simulink model "WBR_Simulator"  (R2023b)
settings: Solver=FixedStepAuto  StartTime=0.0  StopTime=60  FixedStep=0.001  MaxStep=0.001
undefined symbols (not defined in the file or in its folder): DiscIntNeverNeededParam, magnitude, robot_stats, SIMPARAM, X, Y, Z
libraries: sm_lib x73, nesl_utility x50, simulink x17, slpidlib x6, dsparch4 x2
(part 3 of 7)

== system WBR_Simulator/轮子建模 ==
  note: 左轮
  note: 右轮
  左轮控制扭矩 : Inport
  右轮控制扭矩 : Inport  Port=2
  Brick Solid : sm_lib/Body Elements/Brick Solid  GraphicAmbientColor=[0.15 0.15 0.15 1.0]  BasedOnType=Mass  BrickDimensions=[0.1 0.05 0.1]  BrickDimensionsUnits=m  CenterOfMass=[0 0 0]  CenterOfMassUnits=m  GraphicDiffuseColor=[0.5 0.5 0.5]  Density=1000  DensityUnits=kg/m^3  DoExposeReferenceFrame=on  GraphicEmissiveColor=[0.0 0.0 0.0 1.0]  ExportEntireGeometry=off  SerializedFrames=<Frames/>  MarkerShape=Sphere  MarkerSize=10  GraphicType=FromGeometry  InertiaType=CalculateFromGeometry  Mass=0.000001  MassUnits=kg  MomentsOfInertia=[1 1 1]  MomentsOfInertiaUnits=kg*m^2  GraphicOpacity=1.0  ProductsOfInertia=[0 0 0]  ProductsOfInertiaUnits=kg*m^2  GraphicShininess=75  GraphicSpecularColor=[0.5 0.5 0.5 1.0]  GraphicVisPropType=SimpleVisualProperties
  Brick Solid1 : sm_lib/Body Elements/Brick Solid  GraphicAmbientColor=[0.15 0.15 0.15 1.0]  BasedOnType=Mass  BrickDimensions=[0.1 0.05 0.1]  BrickDimensionsUnits=m  CenterOfMass=[0 0 0]  CenterOfMassUnits=m  GraphicDiffuseColor=[0.5 0.5 0.5]  Density=1000  DensityUnits=kg/m^3  DoExposeReferenceFrame=on  GraphicEmissiveColor=[0.0 0.0 0.0 1.0]  ExportEntireGeometry=off  SerializedFrames=<Frames/>  MarkerShape=Sphere  MarkerSize=10  GraphicType=FromGeometry  InertiaType=CalculateFromGeometry  Mass=0.000001  MassUnits=kg  MomentsOfInertia=[1 1 1]  MomentsOfInertiaUnits=kg*m^2  GraphicOpacity=1.0  ProductsOfInertia=[0 0 0]  ProductsOfInertiaUnits=kg*m^2  GraphicShininess=75  GraphicSpecularColor=[0.5 0.5 0.5 1.0]  GraphicVisPropType=SimpleVisualProperties
  Bus Creator3 : BusCreator  Inputs=4
  Cylindrical Solid : sm_lib/Body Elements/Cylindrical Solid  GraphicAmbientColor=[0.15 0.15 0.15 1.0]  BasedOnType=Mass  CenterOfMass=[0 0 0]  CenterOfMassUnits=m  GraphicDiffuseColor=[0.0 0.4 0.4]  CylinderLength=0.05  CylinderLengthUnits=m  CylinderRadius=robot_stats.radius_wheel  CylinderRadiusUnits=m  Density=1000  DensityUnits=kg/m^3  DoExposeReferenceFrame=off  GraphicEmissiveColor=[0.0 0.0 0.0 1.0]  ExportEntireGeometry=on  SerializedFrames=<Frames><Frame><Id>Frame1</Id><Value><Name>center</Name><Origin><Source>GeometricFeature</Source><FeatureName>bottom surface</FeatureName></Origin><PrimaryAxis><DefinedDirection>+Z</DefinedDirection><Source>ReferenceFrame</Source><SourceDirection>+Z</SourceDirection><FeatureName></FeatureName></PrimaryAxis><SecondaryAxis><DefinedDirection>+X</DefinedDirection><Source>ReferenceFrame</Source><SourceDirection>+X</SourceDirection><FeatureName></FeatureName></SecondaryAxis></Value></Frame><Frame><Id>Frame2</Id><Value><Name>F2</Name><Origin><Source>CenterOfMassFrame</Source><FeatureName></FeatureName></Origin><PrimaryAxis><DefinedDirection>+Z</DefinedDirection><Source>ReferenceFrame</Source><SourceDirection>+Z</SourceDirection><FeatureName></FeatureName></PrimaryAxis><SecondaryAxis><DefinedDirection>+X</DefinedDirection><Source>ReferenceFrame</Source><SourceDirection>+X</SourceDirection><FeatureName></FeatureName></SecondaryAxis></Value></Frame></Frames>  MarkerShape=Sphere  MarkerSize=10  GraphicType=FromGeometry  InertiaType=CalculateFromGeometry  Mass=robot_stats.mass_wheel_aver/2  MassUnits=kg  MomentsOfInertia=[1 1 1]  MomentsOfInertiaUnits=kg*m^2  GraphicOpacity=1.0  ProductsOfInertia=[0 0 0]  ProductsOfInertiaUnits=kg*m^2  GraphicShininess=75  GraphicSpecularColor=[0.5 0.5 0.5 1.0]  GraphicVisPropType=SimpleVisualProperties
  Cylindrical Solid1 : sm_lib/Body Elements/Cylindrical Solid  GraphicAmbientColor=[0.15 0.15 0.15 1.0]  BasedOnType=Mass  CenterOfMass=[0 0 0]  CenterOfMassUnits=m  GraphicDiffuseColor=[0.0 0.4 0.4]  CylinderLength=0.05  CylinderLengthUnits=m  CylinderRadius=robot_stats.radius_wheel  CylinderRadiusUnits=m  Density=1000  DensityUnits=kg/m^3  DoExposeReferenceFrame=off  GraphicEmissiveColor=[0.0 0.0 0.0 1.0]  ExportEntireGeometry=on  SerializedFrames=<Frames><Frame><Id>Frame1</Id><Value><Name>center</Name><Origin><Source>GeometricFeature</Source><FeatureName>top surface</FeatureName></Origin><PrimaryAxis><DefinedDirection>+Z</DefinedDirection><Source>ReferenceFrame</Source><SourceDirection>+Z</SourceDirection><FeatureName></FeatureName></PrimaryAxis><SecondaryAxis><DefinedDirection>+X</DefinedDirection><Source>ReferenceFrame</Source><SourceDirection>+X</SourceDirection><FeatureName></FeatureName></SecondaryAxis></Value></Frame><Frame><Id>Frame2</Id><Value><Name>F2</Name><Origin><Source>CenterOfMassFrame</Source><FeatureName></FeatureName></Origin><PrimaryAxis><DefinedDirection>+Z</DefinedDirection><Source>ReferenceFrame</Source><SourceDirection>+Z</SourceDirection><FeatureName></FeatureName></PrimaryAxis><SecondaryAxis><DefinedDirection>+X</DefinedDirection><Source>ReferenceFrame</Source><SourceDirection>+X</SourceDirection><FeatureName></FeatureName></SecondaryAxis></Value></Frame></Frames>  MarkerShape=Sphere  MarkerSize=10  GraphicType=FromGeometry  InertiaType=CalculateFromGeometry  Mass=robot_stats.mass_wheel_aver/2  MassUnits=kg  MomentsOfInertia=[1 1 1]  MomentsOfInertiaUnits=kg*m^2  GraphicOpacity=1.0  ProductsOfInertia=[0 0 0]  ProductsOfInertiaUnits=kg*m^2  GraphicShininess=75  GraphicSpecularColor=[0.5 0.5 0.5 1.0]  GraphicVisPropType=SimpleVisualProperties
  Discrete-Time Integrator : DiscreteIntegrator  SampleTime=-1  ICPrevOutput=DiscIntNeverNeededParam  ICPrevScaledInput=DiscIntNeverNeededParam
  Discrete-Time Integrator1 : DiscreteIntegrator  SampleTime=-1  ICPrevOutput=DiscIntNeverNeededParam  ICPrevScaledInput=DiscIntNeverNeededParam
  Multiply : Gain  Gain=robot_stats.radius_wheel
  Multiply1 : Gain  Gain=robot_stats.radius_wheel
  PS-Simulink Converter : nesl_utility/PS-Simulink Converter  PhysicalDomain=network_engine_domain  SubClassName=ps_output  LeftPortType=input  RightPortType=output  PseudoPeriodic=off  Frequencies=[]  VectorFormat=1-D array  Unit=inherit  AffineConversion=off
  PS-Simulink Converter2 : nesl_utility/PS-Simulink Converter  PhysicalDomain=network_engine_domain  SubClassName=ps_output  LeftPortType=input  RightPortType=output  PseudoPeriodic=off  Frequencies=[]  VectorFormat=1-D array  Unit=inherit  AffineConversion=off
  Revolute Joint2 : sm_lib/Joints/Revolute Joint  JointMode=Normal  SenseConstraintForce=off  SenseConstraintForceX=off  SenseConstraintForceY=off  SenseConstraintForceZ=off  SenseConstraintTorque=off  SenseConstraintTorqueX=off  SenseConstraintTorqueY=off  SenseConstraintTorqueZ=off  SenseTotalForce=off  SenseTotalForceX=off  SenseTotalForceY=off  SenseTotalForceZ=off  SenseTotalTorque=off  SenseTotalTorqueX=off  SenseTotalTorqueY=off  SenseTotalTorqueZ=off  CompositeWrenchDir=FollowerOnBase  CompositeWrenchFrame=BaseFrame  EquilibriumPosition=0  EquilibriumPositionUnits=deg  SpringStiffness=0  SpringStiffnessUnits=N*m/deg  DampingCoefficient=0  DampingCoefficientUnits=N*m/(deg/s)  TorqueActuationMode=InputTorque  MotionActuationMode=ComputedMotion  SensePosition=off  SenseVelocity=on  SenseAcceleration=off  SenseTorqueForce=off  SenseLowerLimitTorqueForce=off  SenseUpperLimitTorqueForce=off  LowerLimitSpecify=off  LowerLimitBound=-90  LowerLimitBoundUnits=deg  LowerLimitStiffness=1e4  LowerLimitStiffnessUnits=N*m/deg  LowerLimitDamping=10  LowerLimitDampingUnits=N*m/(deg/s)  LowerLimitTransitionRegionWidth=0.1  LowerLimitTransitionRegionWidthUnits=deg  UpperLimitSpecify=off  UpperLimitBound=90  UpperLimitBoundUnits=deg  UpperLimitStiffness=1e4  UpperLimitStiffnessUnits=N*m/deg  UpperLimitDamping=10  UpperLimitDampingUnits=N*m/(deg/s)  UpperLimitTransitionRegionWidth=0.1  UpperLimitTransitionRegionWidthUnits=deg  PositionTargetSpecify=on  PositionTargetPriority=High  PositionTargetValue=0  PositionTargetValueUnits=deg  VelocityTargetSpecify=off  VelocityTargetPriority=High  VelocityTargetValue=0  VelocityTargetValueUnits=deg/s
  Revolute Joint7 : sm_lib/Joints/Revolute Joint  JointMode=Normal  SenseConstraintForce=off  SenseConstraintForceX=off  SenseConstraintForceY=off  SenseConstraintForceZ=off  SenseConstraintTorque=off  SenseConstraintTorqueX=off  SenseConstraintTorqueY=off  SenseConstraintTorqueZ=off  SenseTotalForce=off  SenseTotalForceX=off  SenseTotalForceY=off  SenseTotalForceZ=off  SenseTotalTorque=off  SenseTotalTorqueX=off  SenseTotalTorqueY=off  SenseTotalTorqueZ=off  CompositeWrenchDir=FollowerOnBase  CompositeWrenchFrame=BaseFrame  EquilibriumPosition=0  EquilibriumPositionUnits=deg  SpringStiffness=0  SpringStiffnessUnits=N*m/deg  DampingCoefficient=0  DampingCoefficientUnits=N*m/(deg/s)  TorqueActuationMode=InputTorque  MotionActuationMode=ComputedMotion  SensePosition=off  SenseVelocity=on  SenseAcceleration=off  SenseTorqueForce=off  SenseLowerLimitTorqueForce=off  SenseUpperLimitTorqueForce=off  LowerLimitSpecify=off  LowerLimitBound=-90  LowerLimitBoundUnits=deg  LowerLimitStiffness=1e4  LowerLimitStiffnessUnits=N*m/deg  LowerLimitDamping=10  LowerLimitDampingUnits=N*m/(deg/s)  LowerLimitTransitionRegionWidth=0.1  LowerLimitTransitionRegionWidthUnits=deg  UpperLimitSpecify=off  UpperLimitBound=90  UpperLimitBoundUnits=deg  UpperLimitStiffness=1e4  UpperLimitStiffnessUnits=N*m/deg  UpperLimitDamping=10  UpperLimitDampingUnits=N*m/(deg/s)  UpperLimitTransitionRegionWidth=0.1  UpperLimitTransitionRegionWidthUnits=deg  PositionTargetSpecify=on  PositionTargetPriority=High  PositionTargetValue=0  PositionTargetValueUnits=deg  VelocityTargetSpecify=off  VelocityTargetPriority=High  VelocityTargetValue=0  VelocityTargetValueUnits=deg/s
  Rigid Transform : sm_lib/Frames and Transforms/Rigid Transform  TranslationMethod=Cartesian  TranslationStandardOffset=1.5  TranslationStandardOffsetUnits=m  TranslationStandardAxis=-X  TranslationCartesianOffset=[0 0 0]  TranslationCartesianOffsetUnits=m  TranslationROffset=0  TranslationROffsetUnits=m  TranslationZOffset=0  TranslationZOffsetUnits=m  TranslationThetaOffset=0  TranslationThetaOffsetUnits=deg  RotationMethod=StandardAxis  RotationAngleUnits=deg  RotationStandardAxis=+Y  RotationAngle=0  RotationArbitraryAxis=[0 0 1]  FollAlignAxisA=+X  BaseAlignAxisA=+Y  FollAlignAxisB=+Y  BaseAlignAxisB=+Z  RotationSequenceAxes=FollowerAxes  RotationSequence=XYX  RotationSequenceAngles=[0 0 0]  RotationSequenceAnglesUnits=deg  RotationMatrix=[1 0 0; 0 1 0; 0 0 1]  Quaternion=[1 0 0 0]
  Rigid Transform1 : sm_lib/Frames and Transforms/Rigid Transform  TranslationMethod=Cartesian  TranslationStandardOffset=1.5  TranslationStandardOffsetUnits=m  TranslationStandardAxis=-X  TranslationCartesianOffset=[0 0 0]  TranslationCartesianOffsetUnits=m  TranslationROffset=0  TranslationROffsetUnits=m  TranslationZOffset=0  TranslationZOffsetUnits=m  TranslationThetaOffset=0  TranslationThetaOffsetUnits=deg  RotationMethod=StandardAxis  RotationAngleUnits=deg  RotationStandardAxis=+Y  RotationAngle=0  RotationArbitraryAxis=[0 0 1]  FollAlignAxisA=+X  BaseAlignAxisA=+Y  FollAlignAxisB=+Y  BaseAlignAxisB=+Z  RotationSequenceAxes=FollowerAxes  RotationSequence=XYX  RotationSequenceAngles=[0 0 0]  RotationSequenceAnglesUnits=deg  RotationMatrix=[1 0 0; 0 1 0; 0 0 1]  Quaternion=[1 0 0 0]
  Simulink-PS Converter : nesl_utility/Simulink-PS Converter  PhysicalDomain=network_engine_domain  SubClassName=ps_input  LeftPortType=input  RightPortType=output  PseudoPeriodic=off  Frequencies=[]  NoiseDistribution=none  NoiseParameters=[]  Unit=1  AffineConversion=off  FilteringAndDerivatives=provide  SimscapeFilterOrder=1  InputFilterTimeConstant=0.001  UdotUserProvided=0
  Simulink-PS Converter1 : nesl_utility/Simulink-PS Converter  PhysicalDomain=network_engine_domain  SubClassName=ps_input  LeftPortType=input  RightPortType=output  PseudoPeriodic=off  Frequencies=[]  NoiseDistribution=none  NoiseParameters=[]  Unit=1  AffineConversion=off  FilteringAndDerivatives=provide  SimscapeFilterOrder=1  InputFilterTimeConstant=0.001  UdotUserProvided=0
  Spatial Contact Force{,1..3} (4 alike) : sm_lib/Forces and Torques/Spatial Contact Force  SenseContactBaseRotation=off  SenseContactBaseTranslation=off  CoefficientOfDynamicFriction=1  CoefficientOfStaticFriction=1  NormalDamping=1e3  NormalDampingUnits=N/(m/s)  SenseContactSignal=off  NormalStiffness=1e5  NormalStiffnessUnits=N/m  FrictionalCriticalVelocity=1e-3  FrictionalCriticalVelocityUnits=m/s  ZeroCrossDetectContactStartAndEnd=off  SenseContactFollowerRotation=off  SenseContactFollowerTranslation=off  FrictionType=SmoothStickSlip  SenseFrictionalForceMagnitude=off  SenseNormalForceMagnitude=off  NormalForceType=SmoothSpringDamper  SenseNormalVelocity=off  SensePenetrationDepth=off  SenseSeparationDistance=off  SenseTangentialVelocity=off  NormalTransitionRegionWidth=1e-4  NormalTransitionRegionWidthUnits=m
  Zero-Order Hold : ZeroOrderHold  SampleTime=0.001
  Zero-Order Hold1 : ZeroOrderHold  SampleTime=0.001
  左轮坐标系 : PMIOPort  Side=Left
  右轮坐标系 : PMIOPort  Port=2  Side=Left
  轮子地面碰撞 : PMIOPort  Port=3  Side=Left
  轮子飞坡碰撞 : PMIOPort  Port=4  Side=Left
  底盘位置&速度 : Outport
  wires:
  右轮控制扭矩/1 -> Simulink-PS Converter1/1
  左轮控制扭矩/1 -> Simulink-PS Converter/1
  PS-Simulink Converter/1 -> Zero-Order Hold/1
  Multiply/1 -> Discrete-Time Integrator/1, Bus Creator3/2  "v_xl"
  Discrete-Time Integrator/1 -> Bus Creator3/1  "xl"
  Bus Creator3/1 -> 底盘位置&速度/1
  PS-Simulink Converter2/1 -> Zero-Order Hold1/1
  Multiply1/1 -> Discrete-Time Integrator1/1, Bus Creator3/4  "v_xr"
  Discrete-Time Integrator1/1 -> Bus Creator3/3  "xr"
  Zero-Order Hold/1 -> Multiply/1
  Zero-Order Hold1/1 -> Multiply1/1
  connections:
  Simulink-PS Converter/RConn1 -- Revolute Joint7/LConn2
  Spatial Contact Force1/LConn1 -- Spatial Contact Force/LConn1 -- 轮子地面碰撞/RConn1
  Cylindrical Solid1/LConn1 -- Revolute Joint2/RConn1
  Spatial Contact Force2/LConn1 -- Spatial Contact Force3/LConn1 -- 轮子飞坡碰撞/RConn1
  Revolute Joint7/RConn1 -- Cylindrical Solid/LConn1
  Simulink-PS Converter1/RConn1 -- Revolute Joint2/LConn2
  左轮坐标系/RConn1 -- Revolute Joint7/LConn1
  右轮坐标系/RConn1 -- Revolute Joint2/LConn1
  PS-Simulink Converter/LConn1 -- Revolute Joint7/RConn2
  PS-Simulink Converter2/LConn1 -- Revolute Joint2/RConn2
  Spatial Contact Force1/RConn1 -- Cylindrical Solid1/LConn2 -- Spatial Contact Force2/RConn1
  Spatial Contact Force3/RConn1 -- Cylindrical Solid/LConn2 -- Spatial Contact Force/RConn1
  Rigid Transform/RConn1 -- Cylindrical Solid/RConn1
  Brick Solid/RConn1 -- Rigid Transform/LConn1
  Brick Solid1/RConn1 -- Rigid Transform1/LConn1
  Cylindrical Solid1/RConn1 -- Rigid Transform1/RConn1

== system WBR_Simulator/底盘控制器/If Action Subsystem ==
  In1 : Inport
  Action Port : ActionPort  ActionPortLabel=if(u1 < 0.5)
  Out1 : Outport
  wires:
  In1/1 -> Out1/1

== system WBR_Simulator/底盘控制器/If Action Subsystem1 ==
  In1 : Inport
  Action Port : ActionPort  ActionPortLabel=else
  Out1 : Outport
  wires:
  In1/1 -> Out1/1

== system WBR_Simulator/底盘控制器/If Action Subsystem2 ==
  In1 : Inport
  Action Port : ActionPort  ActionPortLabel=if(u1 < 0.5)
  Out1 : Outport
  wires:
  In1/1 -> Out1/1

== system WBR_Simulator/底盘控制器/If Action Subsystem3 ==
  In1 : Inport
  Action Port : ActionPort  ActionPortLabel=else
  Out1 : Outport
  wires:
  In1/1 -> Out1/1

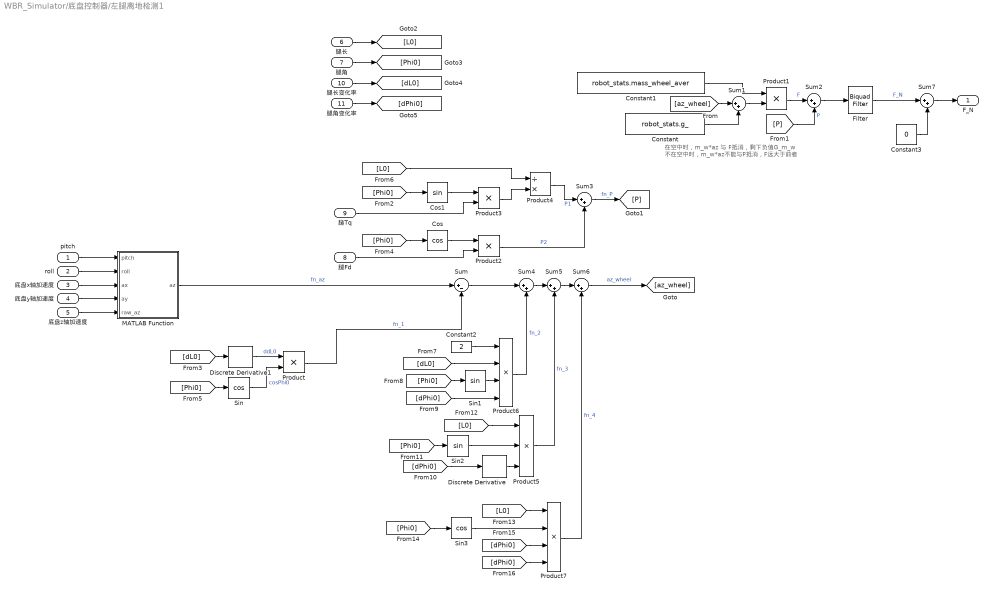
== system WBR_Simulator/底盘控制器/左腿离地检测1 ==
  note: 在空中时，m_w*az 与 P抵消，剩下负值G_m_w
      | 不在空中时，m_w*az不能与P抵消，P远大于前者
  pitch : Inport
  roll : Inport  Port=2
  底盘x轴加速度 : Inport  Port=3
  底盘y轴加速度 : Inport  Port=4
  底盘z轴加速度 : Inport  Port=5
  腿长 : Inport  Port=6
  腿角 : Inport  Port=7
  腿Fd : Inport  Port=8
  腿Tq : Inport  Port=9
  腿长变化率 : Inport  Port=10
  腿角变化率 : Inport  Port=11
  Constant : Constant  Value=robot_stats.g_
  Constant1 : Constant  Value=robot_stats.mass_wheel_aver
  Constant2 : Constant  Value=2
  Constant3 : Constant  Value=0
  Cos : Trigonometry  Operator=cos
  Cos1 : Trigonometry
  Discrete Derivative : simulink/Discrete/Discrete Derivative  gainval=1.0  ICPrevScaledInput=0.0  OutMin=[]  OutMax=[]  OutDataType=fixdt(1, 16)  OutScaling=2^-10  DoSatur=off
  Discrete Derivative1 : simulink/Discrete/Discrete Derivative  gainval=1.0  ICPrevScaledInput=0.0  OutMin=[]  OutMax=[]  OutDataType=fixdt(1, 16)  OutScaling=2^-10  DoSatur=off
  Filter : dsparch4/Biquad Filter  Tag=BlockMethodSubSystem  FilterSource=Dialog parameters  CoeffSource=Specify via dialog  FilterObject=BQF  IIRFiltStruct=Direct form II  BiQuadCoeffs=[1 2 1 1 1.48178412853867525 0.831585910854089061;1 2 1 1 1.27721148327892897 0.578720214976092495;1 2 1 1 1.14298050253990069 0.412801598096188549;1 2 1 1 1.06189684687510155 0.312576687830310729;1 2 1 1 1.0237166685840593 0.265383392069520718]  ScaleValues=[0.828342509848191133;0.713982924563755339;0.638945525159022365;0.593618383676353112;0.572275015163394962;1]  IC=0  ICnum=0  ICden=0  a0Flag=Warning  optimizeScaleValues=on  ScaleValueMode=Specify via input port (g)  InputProcessing=Columns as channels (frame based)  roundingMode=Floor  overflowMode=off  scaleValueFracLength=14  denProdOutputFracLength=30  denAccumFracLength=30  secondMemoryFracLength=15
  MATLAB Function : MATLAB Function  TreatAsAtomicUnit=on
  Product{,1..3} (4 alike) : Product
  Product4 : Product  Inputs=/*
  Product5 : Product  Inputs=3
  Product6 : Product  Inputs=4
  Product7 : Product  Inputs=4
  Sin : Trigonometry  Operator=cos
  Sin1 : Trigonometry
  Sin2 : Trigonometry
  Sin3 : Trigonometry  Operator=cos
  Sum : Sum  Inputs=|+-
  Sum{1..7} (7 alike) : Sum  Inputs=|++
  F_N : Outport
  wires:
  Sin/1 -> Product/2  "cosPhi0"
  Product/1 -> Sum/2  "fn_1"
  [az_wheel] -> Sum1/1
  Constant/1 -> Sum1/2
  Sum1/1 -> Product1/2
  Constant1/1 -> Product1/1
  Product1/1 -> Sum2/1  "F"
  Sum2/1 -> Filter/1
  Cos/1 -> Product2/1
  腿Fd/1 -> Product2/2
  Cos1/1 -> Product3/1
  腿Tq/1 -> Product3/2
  Product2/1 -> Sum3/2  "P2"
  Product4/1 -> Sum3/1  "P1"
  [P] -> Sum2/2  "P"
  腿长/1 -> [L0]
  腿角/1 -> [Phi0]
  [Phi0] -> Cos1/1
  [Phi0] -> Cos/1
  [Phi0] -> Sin/1
  Product3/1 -> Product4/2
  [L0] -> Product4/1
  [dL0] -> Discrete Derivative1/1
  Discrete Derivative1/1 -> Product/1  "ddL0"
  Sum/1 -> Sum4/1
  [Phi0] -> Sin1/1
  腿长变化率/1 -> [dL0]
  腿角变化率/1 -> [dPhi0]
  Sin1/1 -> Product6/3
  [dPhi0] -> Product6/4
  Constant2/1 -> Product6/1
  [dL0] -> Product6/2
  Product6/1 -> Sum4/2  "fn_2"
  [dPhi0] -> Discrete Derivative/1
  Discrete Derivative/1 -> Product5/3
  [Phi0] -> Sin2/1
  Sin2/1 -> Product5/2
  [L0] -> Product5/1
  Sum4/1 -> Sum5/1
  Product5/1 -> Sum5/2  "fn_3"
  Sin3/1 -> Product7/2
  [Phi0] -> Sin3/1
  [L0] -> Product7/1
  [dPhi0] -> Product7/3
  [dPhi0] -> Product7/4
  Sum5/1 -> Sum6/1
  Product7/1 -> Sum6/2  "fn_4"
  Filter/1 -> Sum7/1  "F_N"
  Sum7/1 -> F_N/1
  Constant3/1 -> Sum7/2
  Sum6/1 -> [az_wheel]  "az_wheel"
  pitch/1 -> MATLAB Function/1(pitch)
  roll/1 -> MATLAB Function/2(roll)
  底盘x轴加速度/1 -> MATLAB Function/3(ax)
  底盘y轴加速度/1 -> MATLAB Function/4(ay)
  底盘z轴加速度/1 -> MATLAB Function/5(raw_az)
  MATLAB Function/1(az) -> Sum/1  "fn_az"
  Sum3/1 -> [P]  "fn_P"

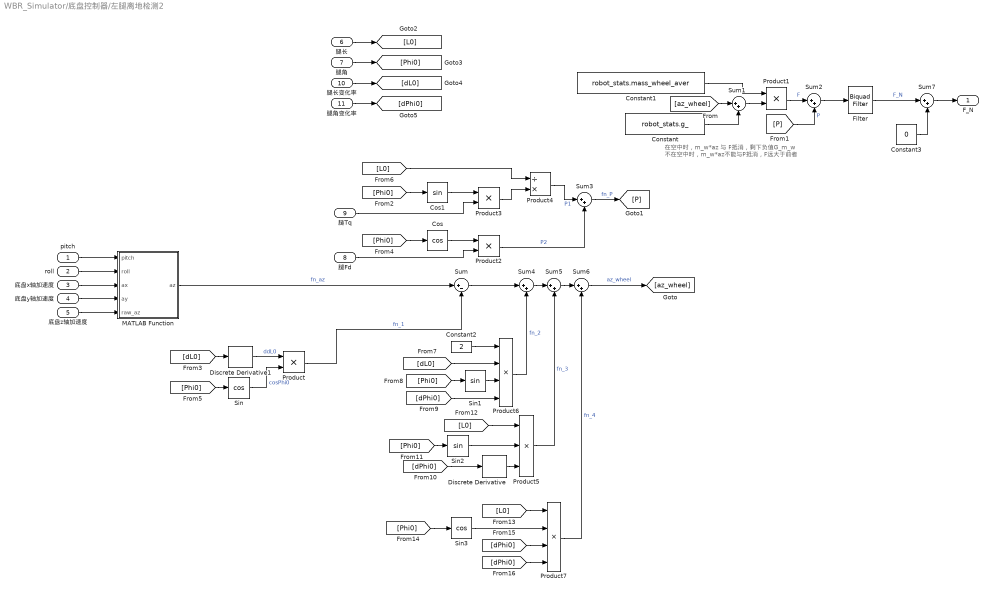
== system WBR_Simulator/底盘控制器/左腿离地检测2 ==
  note: 在空中时，m_w*az 与 P抵消，剩下负值G_m_w
      | 不在空中时，m_w*az不能与P抵消，P远大于前者
  pitch : Inport
  roll : Inport  Port=2
  底盘x轴加速度 : Inport  Port=3
  底盘y轴加速度 : Inport  Port=4
  底盘z轴加速度 : Inport  Port=5
  腿长 : Inport  Port=6
  腿角 : Inport  Port=7
  腿Fd : Inport  Port=8
  腿Tq : Inport  Port=9
  腿长变化率 : Inport  Port=10
  腿角变化率 : Inport  Port=11
  Constant : Constant  Value=robot_stats.g_
  Constant1 : Constant  Value=robot_stats.mass_wheel_aver
  Constant2 : Constant  Value=2
  Constant3 : Constant  Value=0
  Cos : Trigonometry  Operator=cos
  Cos1 : Trigonometry
  Discrete Derivative : simulink/Discrete/Discrete Derivative  gainval=1.0  ICPrevScaledInput=0.0  OutMin=[]  OutMax=[]  OutDataType=fixdt(1, 16)  OutScaling=2^-10  DoSatur=off
  Discrete Derivative1 : simulink/Discrete/Discrete Derivative  gainval=1.0  ICPrevScaledInput=0.0  OutMin=[]  OutMax=[]  OutDataType=fixdt(1, 16)  OutScaling=2^-10  DoSatur=off
  Filter : dsparch4/Biquad Filter  Tag=BlockMethodSubSystem  FilterSource=Dialog parameters  CoeffSource=Specify via dialog  FilterObject=BQF  IIRFiltStruct=Direct form II  BiQuadCoeffs=[1 2 1 1 1.48178412853867525 0.831585910854089061;1 2 1 1 1.27721148327892897 0.578720214976092495;1 2 1 1 1.14298050253990069 0.412801598096188549;1 2 1 1 1.06189684687510155 0.312576687830310729;1 2 1 1 1.0237166685840593 0.265383392069520718]  ScaleValues=[0.828342509848191133;0.713982924563755339;0.638945525159022365;0.593618383676353112;0.572275015163394962;1]  IC=0  ICnum=0  ICden=0  a0Flag=Warning  optimizeScaleValues=on  ScaleValueMode=Specify via input port (g)  InputProcessing=Columns as channels (frame based)  roundingMode=Floor  overflowMode=off  scaleValueFracLength=14  denProdOutputFracLength=30  denAccumFracLength=30  secondMemoryFracLength=15
  MATLAB Function : MATLAB Function  TreatAsAtomicUnit=on
  Product{,1..3} (4 alike) : Product
  Product4 : Product  Inputs=/*
  Product5 : Product  Inputs=3
  Product6 : Product  Inputs=4
  Product7 : Product  Inputs=4
  Sin : Trigonometry  Operator=cos
  Sin1 : Trigonometry
  Sin2 : Trigonometry
  Sin3 : Trigonometry  Operator=cos
  Sum : Sum  Inputs=|+-
  Sum{1..7} (7 alike) : Sum  Inputs=|++
  F_N : Outport
  wires:
  Sin/1 -> Product/2  "cosPhi0"
  Product/1 -> Sum/2  "fn_1"
  [az_wheel] -> Sum1/1
  Constant/1 -> Sum1/2
  Sum1/1 -> Product1/2
  Constant1/1 -> Product1/1
  Product1/1 -> Sum2/1  "F"
  Sum2/1 -> Filter/1
  Cos/1 -> Product2/1
  腿Fd/1 -> Product2/2
  Cos1/1 -> Product3/1
  腿Tq/1 -> Product3/2
  Product2/1 -> Sum3/2  "P2"
  Product4/1 -> Sum3/1  "P1"
  [P] -> Sum2/2  "P"
  腿长/1 -> [L0]
  腿角/1 -> [Phi0]
  [Phi0] -> Cos1/1
  [Phi0] -> Cos/1
  [Phi0] -> Sin/1
  Product3/1 -> Product4/2
  [L0] -> Product4/1
  [dL0] -> Discrete Derivative1/1
  Discrete Derivative1/1 -> Product/1  "ddL0"
  Sum/1 -> Sum4/1
  [Phi0] -> Sin1/1
  腿长变化率/1 -> [dL0]
  腿角变化率/1 -> [dPhi0]
  Sin1/1 -> Product6/3
  [dPhi0] -> Product6/4
  Constant2/1 -> Product6/1
  [dL0] -> Product6/2
  Product6/1 -> Sum4/2  "fn_2"
  [dPhi0] -> Discrete Derivative/1
  Discrete Derivative/1 -> Product5/3
  [Phi0] -> Sin2/1
  Sin2/1 -> Product5/2
  [L0] -> Product5/1
  Sum4/1 -> Sum5/1
  Product5/1 -> Sum5/2  "fn_3"
  Sin3/1 -> Product7/2
  [Phi0] -> Sin3/1
  [L0] -> Product7/1
  [dPhi0] -> Product7/3
  [dPhi0] -> Product7/4
  Sum5/1 -> Sum6/1
  Product7/1 -> Sum6/2  "fn_4"
  Filter/1 -> Sum7/1  "F_N"
  Sum7/1 -> F_N/1
  Constant3/1 -> Sum7/2
  Sum6/1 -> [az_wheel]  "az_wheel"
  pitch/1 -> MATLAB Function/1(pitch)
  roll/1 -> MATLAB Function/2(roll)
  底盘x轴加速度/1 -> MATLAB Function/3(ax)
  底盘y轴加速度/1 -> MATLAB Function/4(ay)
  底盘z轴加速度/1 -> MATLAB Function/5(raw_az)
  MATLAB Function/1(az) -> Sum/1  "fn_az"
  Sum3/1 -> [P]  "fn_P"

== system WBR_Simulator/腿建模/串联腿 ==
  note: 出现过原始角速度跳变的情况
  note: 此处phi0为平行z轴为0,往越往x轴越大
  设定切向力矩 : Inport
  设定径向力 : Inport  Port=2
  Add : Sum
  Brick Solid : sm_lib/Body Elements/Brick Solid  GraphicAmbientColor=[0.15 0.15 0.15 1.0]  BasedOnType=Mass  BrickDimensions=[SIMPARAM.L5 0.01 0.01]  BrickDimensionsUnits=m  CenterOfMass=[0 0 0]  CenterOfMassUnits=m  GraphicDiffuseColor=[0.2 0.0 0.0]  Density=1000  DensityUnits=kg/m^3  DoExposeReferenceFrame=on  GraphicEmissiveColor=[0.0 0.0 0.0 1.0]  ExportEntireGeometry=on  SerializedFrames=<Frames><Frame><Id>Frame2</Id><Value><Name>A</Name><Origin><Source>CenterOfMassFrame</Source><FeatureName></FeatureName></Origin><PrimaryAxis><DefinedDirection>+Y</DefinedDirection><Source>ReferenceFrame</Source><SourceDirection>+Z</SourceDirection><FeatureName></FeatureName></PrimaryAxis><SecondaryAxis><DefinedDirection>+X</DefinedDirection><Source>ReferenceFrame</Source><SourceDirection>+X</SourceDirection><FeatureName></FeatureName></SecondaryAxis></Value></Frame></Frames>  MarkerShape=Sphere  MarkerSize=10  GraphicType=FromGeometry  InertiaType=CalculateFromGeometry  Mass=0.00001  MassUnits=kg  MomentsOfInertia=[1 1 1]  MomentsOfInertiaUnits=kg*m^2  GraphicOpacity=1.0  ProductsOfInertia=[0 0 0]  ProductsOfInertiaUnits=kg*m^2  GraphicShininess=75  GraphicSpecularColor=[0.5 0.5 0.5 1.0]  GraphicVisPropType=SimpleVisualProperties
  Brick Solid1 : sm_lib/Body Elements/Brick Solid  GraphicAmbientColor=[0.15 0.15 0.15 1.0]  BasedOnType=Mass  BrickDimensions=[robot_stats.length_thigh 0.01 0.01]  BrickDimensionsUnits=m  CenterOfMass=[0 0 0]  CenterOfMassUnits=m  GraphicDiffuseColor=[0.0 0.8 1.0]  Density=1000  DensityUnits=kg/m^3  DoExposeReferenceFrame=off  GraphicEmissiveColor=[0.0 0.0 0.0 1.0]  ExportEntireGeometry=off  SerializedFrames=<Frames><Frame><Id>Frame1</Id><Value><Name>A</Name><Origin><Source>GeometricFeature</Source><FeatureName>-x surface</FeatureName></Origin><PrimaryAxis><DefinedDirection>+Y</DefinedDirection><Source>ReferenceFrame</Source><SourceDirection>+Z</SourceDirection><FeatureName></FeatureName></PrimaryAxis><SecondaryAxis><DefinedDirection>+X</DefinedDirection><Source>ReferenceFrame</Source><SourceDirection>+X</SourceDirection><FeatureName></FeatureName></SecondaryAxis></Value></Frame><Frame><Id>Frame2</Id><Value><Name>B</Name><Origin><Source>GeometricFeature</Source><FeatureName>+x surface</FeatureName></Origin><PrimaryAxis><DefinedDirection>+Y</DefinedDirection><Source>ReferenceFrame</Source><SourceDirection>+Z</SourceDirection><FeatureName></FeatureName></PrimaryAxis><SecondaryAxis><DefinedDirection>+X</DefinedDirection><Source>ReferenceFrame</Source><SourceDirection>+X</SourceDirection><FeatureName></FeatureName></SecondaryAxis></Value></Frame></Frames>  MarkerShape=Sphere  MarkerSize=10  GraphicType=FromGeometry  InertiaType=CalculateFromGeometry  Mass=robot_stats.mass_thigh_aver  MassUnits=kg  MomentsOfInertia=[1 1 1]  MomentsOfInertiaUnits=kg*m^2  GraphicOpacity=1.0  ProductsOfInertia=[0 0 0]  ProductsOfInertiaUnits=kg*m^2  GraphicShininess=75  GraphicSpecularColor=[0.5 0.5 0.5 1.0]  GraphicVisPropType=SimpleVisualProperties
  Brick Solid3 : sm_lib/Body Elements/Brick Solid  GraphicAmbientColor=[0.15 0.15 0.15 1.0]  BasedOnType=Mass  BrickDimensions="[robot_stats.length_calf  0.01 0.01]"  BrickDimensionsUnits=m  CenterOfMass=[0 0 0]  CenterOfMassUnits=m  GraphicDiffuseColor=[1.0 0.0 0.0]  Density=1000  DensityUnits=kg/m^3  DoExposeReferenceFrame=off  GraphicEmissiveColor=[0.0 0.0 0.0 1.0]  ExportEntireGeometry=off  SerializedFrames=<Frames><Frame><Id>Frame1</Id><Value><Name>B</Name><Origin><Source>GeometricFeature</Source><FeatureName>-x surface</FeatureName></Origin><PrimaryAxis><DefinedDirection>+Y</DefinedDirection><Source>ReferenceFrame</Source><SourceDirection>+Z</SourceDirection><FeatureName></FeatureName></PrimaryAxis><SecondaryAxis><DefinedDirection>+X</DefinedDirection><Source>ReferenceFrame</Source><SourceDirection>+X</SourceDirection><FeatureName></FeatureName></SecondaryAxis></Value></Frame><Frame><Id>Frame2</Id><Value><Name>C</Name><Origin><Source>GeometricFeature</Source><FeatureName>+x surface</FeatureName></Origin><PrimaryAxis><DefinedDirection>-Y</DefinedDirection><Source>ReferenceFrame</Source><SourceDirection>+Z</SourceDirection><FeatureName></FeatureName></PrimaryAxis><SecondaryAxis><DefinedDirection>+X</DefinedDirection><Source>ReferenceFrame</Source><SourceDirection>+X</SourceDirection><FeatureName></FeatureName></SecondaryAxis></Value></Frame></Frames>  MarkerShape=Sphere  MarkerSize=10  GraphicType=FromGeometry  InertiaType=CalculateFromGeometry  Mass=robot_stats.mass_calf_aver  MassUnits=kg  MomentsOfInertia=[1 1 1]  MomentsOfInertiaUnits=kg*m^2  GraphicOpacity=1.0  ProductsOfInertia=[0 0 0]  ProductsOfInertiaUnits=kg*m^2  GraphicShininess=75  GraphicSpecularColor=[0.5 0.5 0.5 1.0]  GraphicVisPropType=SimpleVisualProperties
  Brick Solid5 : sm_lib/Body Elements/Brick Solid  GraphicAmbientColor=[0.15 0.15 0.15 1.0]  BasedOnType=Mass  BrickDimensions=[0.01 0.01 0.01]  BrickDimensionsUnits=m  CenterOfMass=[0 0 0]  CenterOfMassUnits=m  GraphicDiffuseColor=[0.5 0.5 0.5]  Density=1000  DensityUnits=kg/m^3  DoExposeReferenceFrame=on  GraphicEmissiveColor=[0.0 0.0 0.0 1.0]  ExportEntireGeometry=off  SerializedFrames=<Frames><Frame><Id>Frame1</Id><Value><Name>joint</Name><Origin><Source>CenterOfMassFrame</Source><FeatureName></FeatureName></Origin><PrimaryAxis><DefinedDirection>-Z</DefinedDirection><Source>ReferenceFrame</Source><SourceDirection>+Z</SourceDirection><FeatureName></FeatureName></PrimaryAxis><SecondaryAxis><DefinedDirection>+X</DefinedDirection><Source>ReferenceFrame</Source><SourceDirection>+X</SourceDirection><FeatureName></FeatureName></SecondaryAxis></Value></Frame></Frames>  MarkerShape=Sphere  MarkerSize=10  GraphicType=FromGeometry  InertiaType=CalculateFromGeometry  Mass=0.00001  MassUnits=kg  MomentsOfInertia=[1 1 1]  MomentsOfInertiaUnits=kg*m^2  GraphicOpacity=1.0  ProductsOfInertia=[0 0 0]  ProductsOfInertiaUnits=kg*m^2  GraphicShininess=75  GraphicSpecularColor=[0.5 0.5 0.5 1.0]  GraphicVisPropType=SimpleVisualProperties
  Bus Creator : BusCreator  Inputs=4
  Bus Creator1 : BusCreator  Inputs=2
  Bus Creator6 : BusCreator  Inputs=2
  Bus Selector : BusSelector  OutputSignals=phi_1,phi_2
  Bus Selector1 : BusSelector  OutputSignals=phi_1,phi_2,wphi_1,wphi_2
  Connection Label1 : ConnectionLabel  Label=base_frame
  Connection Label6 : ConnectionLabel  Label=base_frame
  Multiply : Gain
  PS-Simulink Converter{,1..3} (4 alike) : nesl_utility/PS-Simulink Converter  PhysicalDomain=network_engine_domain  SubClassName=ps_output  LeftPortType=input  RightPortType=output  PseudoPeriodic=off  Frequencies=[]  VectorFormat=1-D array  Unit=inherit  AffineConversion=off
  Revolute Joint : sm_lib/Joints/Revolute Joint  JointMode=Normal  SenseConstraintForce=off  SenseConstraintForceX=off  SenseConstraintForceY=off  SenseConstraintForceZ=off  SenseConstraintTorque=off  SenseConstraintTorqueX=off  SenseConstraintTorqueY=off  SenseConstraintTorqueZ=off  SenseTotalForce=off  SenseTotalForceX=off  SenseTotalForceY=off  SenseTotalForceZ=off  SenseTotalTorque=off  SenseTotalTorqueX=off  SenseTotalTorqueY=off  SenseTotalTorqueZ=off  CompositeWrenchDir=FollowerOnBase  CompositeWrenchFrame=BaseFrame  EquilibriumPosition=0  EquilibriumPositionUnits=deg  SpringStiffness=0  SpringStiffnessUnits=N*m/deg  DampingCoefficient=0  DampingCoefficientUnits=N*m/(deg/s)  TorqueActuationMode=InputTorque  MotionActuationMode=ComputedMotion  SensePosition=on  SenseVelocity=on  SenseAcceleration=off  SenseTorqueForce=off  SenseLowerLimitTorqueForce=off  SenseUpperLimitTorqueForce=off  LowerLimitSpecify=off  LowerLimitBound=-90  LowerLimitBoundUnits=deg  LowerLimitStiffness=1e4  LowerLimitStiffnessUnits=N*m/deg  LowerLimitDamping=10  LowerLimitDampingUnits=N*m/(deg/s)  LowerLimitTransitionRegionWidth=0.1  LowerLimitTransitionRegionWidthUnits=deg  UpperLimitSpecify=off  UpperLimitBound=90  UpperLimitBoundUnits=deg  UpperLimitStiffness=1e4  UpperLimitStiffnessUnits=N*m/deg  UpperLimitDamping=10  UpperLimitDampingUnits=N*m/(deg/s)  UpperLimitTransitionRegionWidth=0.1  UpperLimitTransitionRegionWidthUnits=deg  PositionTargetSpecify=on  PositionTargetPriority=High  PositionTargetValue=SIMPARAM.init_phi1  PositionTargetValueUnits=rad  VelocityTargetSpecify=off  VelocityTargetPriority=High  VelocityTargetValue=0  VelocityTargetValueUnits=deg/s
  Revolute Joint2 : sm_lib/Joints/Revolute Joint  JointMode=Normal  SenseConstraintForce=off  SenseConstraintForceX=off  SenseConstraintForceY=off  SenseConstraintForceZ=off  SenseConstraintTorque=off  SenseConstraintTorqueX=off  SenseConstraintTorqueY=off  SenseConstraintTorqueZ=off  SenseTotalForce=off  SenseTotalForceX=off  SenseTotalForceY=off  SenseTotalForceZ=off  SenseTotalTorque=off  SenseTotalTorqueX=off  SenseTotalTorqueY=off  SenseTotalTorqueZ=off  CompositeWrenchDir=FollowerOnBase  CompositeWrenchFrame=BaseFrame  EquilibriumPosition=0  EquilibriumPositionUnits=deg  SpringStiffness=0  SpringStiffnessUnits=N*m/deg  DampingCoefficient=0  DampingCoefficientUnits=N*m/(deg/s)  TorqueActuationMode=InputTorque  MotionActuationMode=ComputedMotion  SensePosition=on  SenseVelocity=on  SenseAcceleration=off  SenseTorqueForce=off  SenseLowerLimitTorqueForce=off  SenseUpperLimitTorqueForce=off  LowerLimitSpecify=off  LowerLimitBound=-90  LowerLimitBoundUnits=deg  LowerLimitStiffness=1e4  LowerLimitStiffnessUnits=N*m/deg  LowerLimitDamping=10  LowerLimitDampingUnits=N*m/(deg/s)  LowerLimitTransitionRegionWidth=0.1  LowerLimitTransitionRegionWidthUnits=deg  UpperLimitSpecify=off  UpperLimitBound=90  UpperLimitBoundUnits=deg  UpperLimitStiffness=1e4  UpperLimitStiffnessUnits=N*m/deg  UpperLimitDamping=10  UpperLimitDampingUnits=N*m/(deg/s)  UpperLimitTransitionRegionWidth=0.1  UpperLimitTransitionRegionWidthUnits=deg  PositionTargetSpecify=on  PositionTargetPriority=High  PositionTargetValue=(SIMPARAM.init_phi2-SIMPARAM.init_phi1)  PositionTargetValueUnits=rad  VelocityTargetSpecify=off  VelocityTargetPriority=High  VelocityTargetValue=0  VelocityTargetValueUnits=deg/s
  Simulink-PS Converter : nesl_utility/Simulink-PS Converter  PhysicalDomain=network_engine_domain  SubClassName=ps_input  LeftPortType=input  RightPortType=output  PseudoPeriodic=off  Frequencies=[]  NoiseDistribution=none  NoiseParameters=[]  Unit=1  AffineConversion=off  FilteringAndDerivatives=provide  SimscapeFilterOrder=1  InputFilterTimeConstant=0.001  UdotUserProvided=0
  Simulink-PS Converter1 : nesl_utility/Simulink-PS Converter  PhysicalDomain=network_engine_domain  SubClassName=ps_input  LeftPortType=input  RightPortType=output  PseudoPeriodic=off  Frequencies=[]  NoiseDistribution=none  NoiseParameters=[]  Unit=1  AffineConversion=off  FilteringAndDerivatives=provide  SimscapeFilterOrder=1  InputFilterTimeConstant=0.001  UdotUserProvided=0
  Spatial Contact Force2 : sm_lib/Forces and Torques/Spatial Contact Force  SenseContactBaseRotation=off  SenseContactBaseTranslation=off  CoefficientOfDynamicFriction=0.3  CoefficientOfStaticFriction=0.5  NormalDamping=1e6  NormalDampingUnits=N/(m/s)  SenseContactSignal=off  NormalStiffness=1e6  NormalStiffnessUnits=N/m  FrictionalCriticalVelocity=1e-3  FrictionalCriticalVelocityUnits=m/s  ZeroCrossDetectContactStartAndEnd=off  SenseContactFollowerRotation=off  SenseContactFollowerTranslation=off  FrictionType=SmoothStickSlip  SenseFrictionalForceMagnitude=off  SenseNormalForceMagnitude=off  NormalForceType=SmoothSpringDamper  SenseNormalVelocity=off  SensePenetrationDepth=off  SenseSeparationDistance=off  SenseTangentialVelocity=off  NormalTransitionRegionWidth=1e-4  NormalTransitionRegionWidthUnits=m
  Spatial Contact Force7 : sm_lib/Forces and Torques/Spatial Contact Force  SenseContactBaseRotation=off  SenseContactBaseTranslation=off  CoefficientOfDynamicFriction=0.3  CoefficientOfStaticFriction=0.5  NormalDamping=1e6  NormalDampingUnits=N/(m/s)  SenseContactSignal=off  NormalStiffness=1e6  NormalStiffnessUnits=N/m  FrictionalCriticalVelocity=1e-3  FrictionalCriticalVelocityUnits=m/s  ZeroCrossDetectContactStartAndEnd=off  SenseContactFollowerRotation=off  SenseContactFollowerTranslation=off  FrictionType=SmoothStickSlip  SenseFrictionalForceMagnitude=off  SenseNormalForceMagnitude=off  NormalForceType=SmoothSpringDamper  SenseNormalVelocity=off  SensePenetrationDepth=off  SenseSeparationDistance=off  SenseTangentialVelocity=off  NormalTransitionRegionWidth=1e-4  NormalTransitionRegionWidthUnits=m
  Zero-Order Hold{1..4} (4 alike) : ZeroOrderHold  SampleTime=0.001
  五连杆正解算矩阵(关节转至末端) : Subsystem
  腿末端控制器 : Subsystem
  运动学解算验证(仅可证明旋转矩阵 : Subsystem  Commented=on
  基坐标 : PMIOPort  Side=Left
  轮毂坐标轴 : PMIOPort  Port=2  Side=Left
  底盘地面碰撞 : PMIOPort  Port=3  Side=Right
  底盘飞坡碰撞 : PMIOPort  Port=4  Side=Right
  phi_0 : Outport
  L_0 : Outport  Port=2
  real_vq : Outport  Port=3
  real_vd : Outport  Port=4
  valid_tqd : Outport  Port=5
  wires:
  腿末端控制器/3(R) -> [R]
  Bus Creator/1 -> Bus Selector/1, Bus Selector1/1
  五连杆正解算矩阵(关节转至末端)/1(J) -> 腿末端控制器/6(J)  "J矩阵"
  腿末端控制器/4(R_inv) -> [R_inv]
  [R_inv] -> 运动学解算验证(仅可证明旋转矩阵/2(R_inv)
  [R] -> 运动学解算验证(仅可证明旋转矩阵/1(R)
  Bus Creator1/1 -> ?  "关节扭矩"
  腿末端控制器/5(phi_0) -> phi_0/1
  腿末端控制器/6(L_0) -> L_0/1
  腿末端控制器/8(real_vd) -> real_vd/1
  腿末端控制器/7(real_vq) -> real_vq/1
  设定切向力矩/1 -> 腿末端控制器/4(set_tq)
  设定径向力/1 -> 腿末端控制器/5(set_fd)
  PS-Simulink Converter/1 -> Zero-Order Hold1/1
  PS-Simulink Converter1/1 -> Zero-Order Hold2/1  "phi_2_world"
  腿末端控制器/1(torque_1) -> Bus Creator1/1, Simulink-PS Converter/1
  腿末端控制器/2(torque_2) -> Bus Creator1/2, Multiply/1
  PS-Simulink Converter2/1 -> Zero-Order Hold3/1
  PS-Simulink Converter3/1 -> Zero-Order Hold4/1
  腿末端控制器/9(valid_tqd) -> valid_tqd/1
  Bus Creator6/1 -> 腿末端控制器/1(phi)
  Add/1 -> Bus Creator/2  "phi_2"
  Bus Selector/1 -> 五连杆正解算矩阵(关节转至末端)/1(phi_1)  "<phi_1>"
  Bus Selector/2 -> 五连杆正解算矩阵(关节转至末端)/2(phi_2)  "<phi_2>"
  Bus Selector1/1 -> Bus Creator6/1  "<phi_1>"
  Bus Selector1/2 -> Bus Creator6/2  "<phi_2>"
  Bus Selector1/3 -> 腿末端控制器/2(wphi_1)  "<wphi_1>"
  Bus Selector1/4 -> 腿末端控制器/3(wphi_2)  "<wphi_2>"
  Multiply/1 -> Simulink-PS Converter1/1
  Zero-Order Hold1/1 -> Add/1, Bus Creator/1  "phi_1"
  Zero-Order Hold2/1 -> Add/2
  Zero-Order Hold3/1 -> Bus Creator/3  "wphi_1"
  Zero-Order Hold4/1 -> Bus Creator/4  "wphi_2"
  connections:
  Revolute Joint2/RConn1 -- Brick Solid3/LConn1
  Revolute Joint/LConn1 -- Brick Solid/LConn1
  Revolute Joint/RConn2 -- PS-Simulink Converter/LConn1
  Revolute Joint/RConn1 -- Brick Solid1/LConn1
  Brick Solid5/RConn1 -- Brick Solid3/RConn1 -- 运动学解算验证(仅可证明旋转矩阵/RConn1
  Revolute Joint/RConn3 -- PS-Simulink Converter2/LConn1
  Connection Label6/LConn1 -- 运动学解算验证(仅可证明旋转矩阵/LConn1
  Brick Solid/RConn1 -- Connection Label1/LConn1 -- 基坐标/RConn1
  Revolute Joint/LConn2 -- Simulink-PS Converter/RConn1
  Simulink-PS Converter1/RConn1 -- Revolute Joint2/LConn2
  Brick Solid5/LConn1 -- 轮毂坐标轴/RConn1
  Brick Solid1/RConn1 -- Revolute Joint2/LConn1
  Spatial Contact Force2/LConn1 -- 底盘地面碰撞/RConn1
  Spatial Contact Force7/RConn1 -- Brick Solid/LConn2 -- Spatial Contact Force2/RConn1
  Spatial Contact Force7/LConn1 -- 底盘飞坡碰撞/RConn1
  Revolute Joint2/RConn3 -- PS-Simulink Converter3/LConn1
  Revolute Joint2/RConn2 -- PS-Simulink Converter1/LConn1
